simulink model "chip_route_iso_mdl"  (R2025b)
settings: Solver=VariableStepAuto  StartTime=0.0  StopTime=10.0  RelTol=1e-3
libraries: fl_lib x62, nesl_utility x1
settings Model: Creator=97638  LastModifiedBy=97638

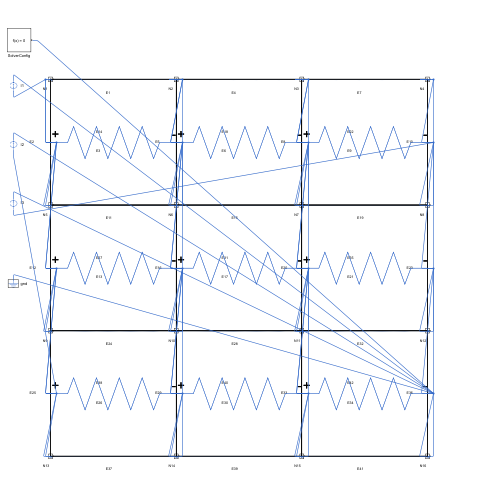
[thumbnail: Simulink's stored preview of the top-level diagram]
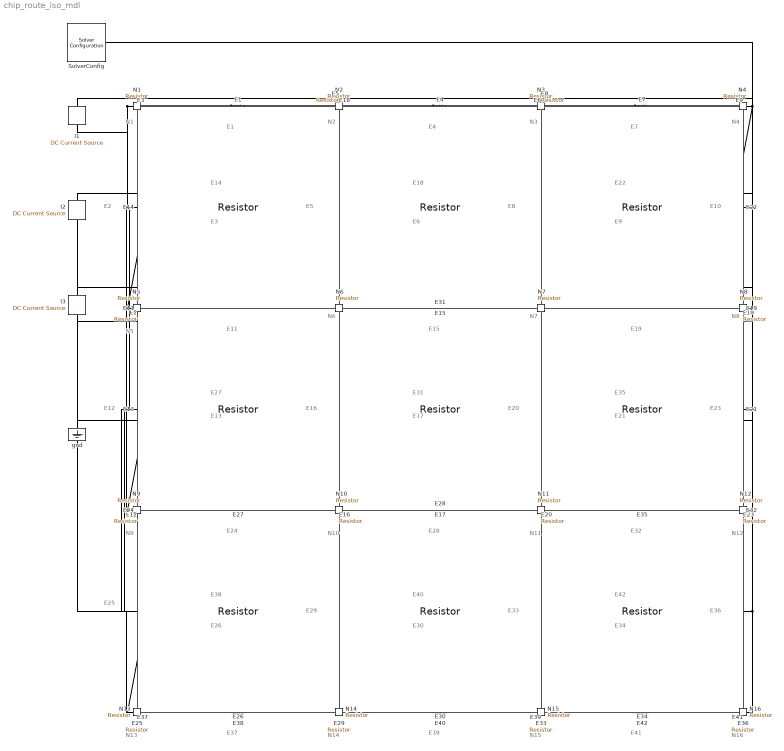
== system chip_route_iso_mdl ==
  note: N1
  note: N2
  note: N3
  note: N4
  note: N5
  note: N6
  note: N7
  note: N8
  note: N9
  note: N10
  note: N11
  note: N12
  note: N13
  note: N14
  note: N15
  note: N16
  note: E1
  note: E2
  note: E3
  note: E4
  note: E5
  note: E6
  note: E7
  note: E8
  note: E9
  note: E10
  note: E11
  note: E12
  note: E13
  note: E14
  note: E15
  note: E16
  note: E17
  note: E18
  note: E19
  note: E20
  note: E21
  note: E22
  note: E23
  note: E24
  note: E25
  note: E26
  note: E27
  note: E28
  note: E29
  note: E30
  note: E31
  note: E32
  note: E33
  note: E34
  note: E35
  note: E36
  note: E37
  note: E38
  note: E39
  note: E40
  note: E41
  note: E42
  E{1..2,4..5,7..8,10..12,15..16,19..20,23..25,28..29,32..33,36..37,39,41} (24 alike) : fl_lib/Electrical/Electrical Elements/Resistor  R=1.000000 Ohm  i_specify=off  i_priority=None  i=0 A  i_nominal_specify=off  i_nominal_value=1  i_nominal_unit=A  v_specify=off  v_priority=None  v=0 V  v_nominal_specify=off  v_nominal_value=1  v_nominal_unit=V  mask(Resistor){}
      E1 mask Display:
      | line([0.0000,0.2500],[0.5000,0.5000]);
      | line([0.2500,0.3125,0.3750,0.4375,0.5000,0.5625,0.6250,0.6875,0.7500],[0.5000,0.4000,0.6000,0.4000,0.6000,0.4000,0.6000,0.4000,0.5000]);
      | line([0.7500,1.0000],[0.5000,0.5000]);
      E10 mask Display:
      | line([0.5000,0.5000],[0.0000,0.2500]);
      | line([0.5000,0.6000,0.4000,0.6000,0.4000,0.6000,0.4000,0.6000,0.5000],[0.2500,0.3125,0.3750,0.4375,0.5000,0.5625,0.6250,0.6875,0.7500]);
      | line([0.5000,0.5000],[0.7500,1.0000]);
      E11 mask Display:
      | line([0.0000,0.2500],[0.5000,0.5000]);
      | line([0.2500,0.3125,0.3750,0.4375,0.5000,0.5625,0.6250,0.6875,0.7500],[0.5000,0.4000,0.6000,0.4000,0.6000,0.4000,0.6000,0.4000,0.5000]);
      | line([0.7500,1.0000],[0.5000,0.5000]);
      E12 mask Display:
      | line([0.5000,0.5000],[0.0000,0.2500]);
      | line([0.5000,0.6000,0.4000,0.6000,0.4000,0.6000,0.4000,0.6000,0.5000],[0.2500,0.3125,0.3750,0.4375,0.5000,0.5625,0.6250,0.6875,0.7500]);
      | line([0.5000,0.5000],[0.7500,1.0000]);
      E15 mask Display:
      | line([0.0000,0.2500],[0.5000,0.5000]);
      | line([0.2500,0.3125,0.3750,0.4375,0.5000,0.5625,0.6250,0.6875,0.7500],[0.5000,0.4000,0.6000,0.4000,0.6000,0.4000,0.6000,0.4000,0.5000]);
      | line([0.7500,1.0000],[0.5000,0.5000]);
      E16 mask Display:
      | line([0.5000,0.5000],[0.0000,0.2500]);
      | line([0.5000,0.6000,0.4000,0.6000,0.4000,0.6000,0.4000,0.6000,0.5000],[0.2500,0.3125,0.3750,0.4375,0.5000,0.5625,0.6250,0.6875,0.7500]);
      | line([0.5000,0.5000],[0.7500,1.0000]);
      E19 mask Display:
      | line([0.0000,0.2500],[0.5000,0.5000]);
      | line([0.2500,0.3125,0.3750,0.4375,0.5000,0.5625,0.6250,0.6875,0.7500],[0.5000,0.4000,0.6000,0.4000,0.6000,0.4000,0.6000,0.4000,0.5000]);
      | line([0.7500,1.0000],[0.5000,0.5000]);
      E2 mask Display:
      | line([0.5000,0.5000],[0.0000,0.2500]);
      | line([0.5000,0.6000,0.4000,0.6000,0.4000,0.6000,0.4000,0.6000,0.5000],[0.2500,0.3125,0.3750,0.4375,0.5000,0.5625,0.6250,0.6875,0.7500]);
      | line([0.5000,0.5000],[0.7500,1.0000]);
      E20 mask Display:
      | line([0.5000,0.5000],[0.0000,0.2500]);
      | line([0.5000,0.6000,0.4000,0.6000,0.4000,0.6000,0.4000,0.6000,0.5000],[0.2500,0.3125,0.3750,0.4375,0.5000,0.5625,0.6250,0.6875,0.7500]);
      | line([0.5000,0.5000],[0.7500,1.0000]);
      E23 mask Display:
      | line([0.5000,0.5000],[0.0000,0.2500]);
      | line([0.5000,0.6000,0.4000,0.6000,0.4000,0.6000,0.4000,0.6000,0.5000],[0.2500,0.3125,0.3750,0.4375,0.5000,0.5625,0.6250,0.6875,0.7500]);
      | line([0.5000,0.5000],[0.7500,1.0000]);
      E24 mask Display:
      | line([0.0000,0.2500],[0.5000,0.5000]);
      | line([0.2500,0.3125,0.3750,0.4375,0.5000,0.5625,0.6250,0.6875,0.7500],[0.5000,0.4000,0.6000,0.4000,0.6000,0.4000,0.6000,0.4000,0.5000]);
      | line([0.7500,1.0000],[0.5000,0.5000]);
      E25 mask Display:
      | line([0.5000,0.5000],[0.0000,0.2500]);
      | line([0.5000,0.6000,0.4000,0.6000,0.4000,0.6000,0.4000,0.6000,0.5000],[0.2500,0.3125,0.3750,0.4375,0.5000,0.5625,0.6250,0.6875,0.7500]);
      | line([0.5000,0.5000],[0.7500,1.0000]);
      E28 mask Display:
      | line([0.0000,0.2500],[0.5000,0.5000]);
      | line([0.2500,0.3125,0.3750,0.4375,0.5000,0.5625,0.6250,0.6875,0.7500],[0.5000,0.4000,0.6000,0.4000,0.6000,0.4000,0.6000,0.4000,0.5000]);
      | line([0.7500,1.0000],[0.5000,0.5000]);
      E29 mask Display:
      | line([0.5000,0.5000],[0.0000,0.2500]);
      | line([0.5000,0.6000,0.4000,0.6000,0.4000,0.6000,0.4000,0.6000,0.5000],[0.2500,0.3125,0.3750,0.4375,0.5000,0.5625,0.6250,0.6875,0.7500]);
      | line([0.5000,0.5000],[0.7500,1.0000]);
      E32 mask Display:
      | line([0.0000,0.2500],[0.5000,0.5000]);
      | line([0.2500,0.3125,0.3750,0.4375,0.5000,0.5625,0.6250,0.6875,0.7500],[0.5000,0.4000,0.6000,0.4000,0.6000,0.4000,0.6000,0.4000,0.5000]);
      | line([0.7500,1.0000],[0.5000,0.5000]);
      E33 mask Display:
      | line([0.5000,0.5000],[0.0000,0.2500]);
      | line([0.5000,0.6000,0.4000,0.6000,0.4000,0.6000,0.4000,0.6000,0.5000],[0.2500,0.3125,0.3750,0.4375,0.5000,0.5625,0.6250,0.6875,0.7500]);
      | line([0.5000,0.5000],[0.7500,1.0000]);
      E36 mask Display:
      | line([0.5000,0.5000],[0.0000,0.2500]);
      | line([0.5000,0.6000,0.4000,0.6000,0.4000,0.6000,0.4000,0.6000,0.5000],[0.2500,0.3125,0.3750,0.4375,0.5000,0.5625,0.6250,0.6875,0.7500]);
      | line([0.5000,0.5000],[0.7500,1.0000]);
      E37 mask Display:
      | line([0.0000,0.2500],[0.5000,0.5000]);
      | line([0.2500,0.3125,0.3750,0.4375,0.5000,0.5625,0.6250,0.6875,0.7500],[0.5000,0.4000,0.6000,0.4000,0.6000,0.4000,0.6000,0.4000,0.5000]);
      | line([0.7500,1.0000],[0.5000,0.5000]);
      E39 mask Display:
      | line([0.0000,0.2500],[0.5000,0.5000]);
      | line([0.2500,0.3125,0.3750,0.4375,0.5000,0.5625,0.6250,0.6875,0.7500],[0.5000,0.4000,0.6000,0.4000,0.6000,0.4000,0.6000,0.4000,0.5000]);
      | line([0.7500,1.0000],[0.5000,0.5000]);
      E4 mask Display:
      | line([0.0000,0.2500],[0.5000,0.5000]);
      | line([0.2500,0.3125,0.3750,0.4375,0.5000,0.5625,0.6250,0.6875,0.7500],[0.5000,0.4000,0.6000,0.4000,0.6000,0.4000,0.6000,0.4000,0.5000]);
      | line([0.7500,1.0000],[0.5000,0.5000]);
      E41 mask Display:
      | line([0.0000,0.2500],[0.5000,0.5000]);
      | line([0.2500,0.3125,0.3750,0.4375,0.5000,0.5625,0.6250,0.6875,0.7500],[0.5000,0.4000,0.6000,0.4000,0.6000,0.4000,0.6000,0.4000,0.5000]);
      | line([0.7500,1.0000],[0.5000,0.5000]);
      E5 mask Display:
      | line([0.5000,0.5000],[0.0000,0.2500]);
      | line([0.5000,0.6000,0.4000,0.6000,0.4000,0.6000,0.4000,0.6000,0.5000],[0.2500,0.3125,0.3750,0.4375,0.5000,0.5625,0.6250,0.6875,0.7500]);
      | line([0.5000,0.5000],[0.7500,1.0000]);
      E7 mask Display:
      | line([0.0000,0.2500],[0.5000,0.5000]);
      | line([0.2500,0.3125,0.3750,0.4375,0.5000,0.5625,0.6250,0.6875,0.7500],[0.5000,0.4000,0.6000,0.4000,0.6000,0.4000,0.6000,0.4000,0.5000]);
      | line([0.7500,1.0000],[0.5000,0.5000]);
      E8 mask Display:
      | line([0.5000,0.5000],[0.0000,0.2500]);
      | line([0.5000,0.6000,0.4000,0.6000,0.4000,0.6000,0.4000,0.6000,0.5000],[0.2500,0.3125,0.3750,0.4375,0.5000,0.5625,0.6250,0.6875,0.7500]);
      | line([0.5000,0.5000],[0.7500,1.0000]);
  E{3,6,9,13..14,17..18,21..22,26..27,30..31,34..35,38,40,42} (18 alike) : fl_lib/Electrical/Electrical Elements/Resistor  R=1.414214 Ohm  i_specify=off  i_priority=None  i=0 A  i_nominal_specify=off  i_nominal_value=1  i_nominal_unit=A  v_specify=off  v_priority=None  v=0 V  v_nominal_specify=off  v_nominal_value=1  v_nominal_unit=V  mask(Resistor){}
      E13 mask Display:
      | line([0.0000,0.2500],[0.0000,0.2500]);
      | line([0.2500,0.3832,0.3043,0.5082,0.4293,0.6332,0.5543,0.7582,0.7500],[0.2500,0.2418,0.4457,0.3668,0.5707,0.4918,0.6957,0.6168,0.7500]);
      | line([0.7500,1.0000],[0.7500,1.0000]);
      E14 mask Display:
      | line([0.0000,0.2500],[1.0000,0.7500]);
      | line([0.2500,0.2418,0.4457,0.3668,0.5707,0.4918,0.6957,0.6168,0.7500],[0.7500,0.6168,0.6957,0.4918,0.5707,0.3668,0.4457,0.2418,0.2500]);
      | line([0.7500,1.0000],[0.2500,0.0000]);
      E17 mask Display:
      | line([0.0000,0.2500],[0.0000,0.2500]);
      | line([0.2500,0.3832,0.3043,0.5082,0.4293,0.6332,0.5543,0.7582,0.7500],[0.2500,0.2418,0.4457,0.3668,0.5707,0.4918,0.6957,0.6168,0.7500]);
      | line([0.7500,1.0000],[0.7500,1.0000]);
      E18 mask Display:
      | line([0.0000,0.2500],[1.0000,0.7500]);
      | line([0.2500,0.2418,0.4457,0.3668,0.5707,0.4918,0.6957,0.6168,0.7500],[0.7500,0.6168,0.6957,0.4918,0.5707,0.3668,0.4457,0.2418,0.2500]);
      | line([0.7500,1.0000],[0.2500,0.0000]);
      E21 mask Display:
      | line([0.0000,0.2500],[0.0000,0.2500]);
      | line([0.2500,0.3832,0.3043,0.5082,0.4293,0.6332,0.5543,0.7582,0.7500],[0.2500,0.2418,0.4457,0.3668,0.5707,0.4918,0.6957,0.6168,0.7500]);
      | line([0.7500,1.0000],[0.7500,1.0000]);
      E22 mask Display:
      | line([0.0000,0.2500],[1.0000,0.7500]);
      | line([0.2500,0.2418,0.4457,0.3668,0.5707,0.4918,0.6957,0.6168,0.7500],[0.7500,0.6168,0.6957,0.4918,0.5707,0.3668,0.4457,0.2418,0.2500]);
      | line([0.7500,1.0000],[0.2500,0.0000]);
      E26 mask Display:
      | line([0.0000,0.2500],[0.0000,0.2500]);
      | line([0.2500,0.3832,0.3043,0.5082,0.4293,0.6332,0.5543,0.7582,0.7500],[0.2500,0.2418,0.4457,0.3668,0.5707,0.4918,0.6957,0.6168,0.7500]);
      | line([0.7500,1.0000],[0.7500,1.0000]);
      E27 mask Display:
      | line([0.0000,0.2500],[1.0000,0.7500]);
      | line([0.2500,0.2418,0.4457,0.3668,0.5707,0.4918,0.6957,0.6168,0.7500],[0.7500,0.6168,0.6957,0.4918,0.5707,0.3668,0.4457,0.2418,0.2500]);
      | line([0.7500,1.0000],[0.2500,0.0000]);
      E3 mask Display:
      | line([0.0000,0.2500],[0.0000,0.2500]);
      | line([0.2500,0.3832,0.3043,0.5082,0.4293,0.6332,0.5543,0.7582,0.7500],[0.2500,0.2418,0.4457,0.3668,0.5707,0.4918,0.6957,0.6168,0.7500]);
      | line([0.7500,1.0000],[0.7500,1.0000]);
      E30 mask Display:
      | line([0.0000,0.2500],[0.0000,0.2500]);
      | line([0.2500,0.3832,0.3043,0.5082,0.4293,0.6332,0.5543,0.7582,0.7500],[0.2500,0.2418,0.4457,0.3668,0.5707,0.4918,0.6957,0.6168,0.7500]);
      | line([0.7500,1.0000],[0.7500,1.0000]);
      E31 mask Display:
      | line([0.0000,0.2500],[1.0000,0.7500]);
      | line([0.2500,0.2418,0.4457,0.3668,0.5707,0.4918,0.6957,0.6168,0.7500],[0.7500,0.6168,0.6957,0.4918,0.5707,0.3668,0.4457,0.2418,0.2500]);
      | line([0.7500,1.0000],[0.2500,0.0000]);
      E34 mask Display:
      | line([0.0000,0.2500],[0.0000,0.2500]);
      | line([0.2500,0.3832,0.3043,0.5082,0.4293,0.6332,0.5543,0.7582,0.7500],[0.2500,0.2418,0.4457,0.3668,0.5707,0.4918,0.6957,0.6168,0.7500]);
      | line([0.7500,1.0000],[0.7500,1.0000]);
      E35 mask Display:
      | line([0.0000,0.2500],[1.0000,0.7500]);
      | line([0.2500,0.2418,0.4457,0.3668,0.5707,0.4918,0.6957,0.6168,0.7500],[0.7500,0.6168,0.6957,0.4918,0.5707,0.3668,0.4457,0.2418,0.2500]);
      | line([0.7500,1.0000],[0.2500,0.0000]);
      E38 mask Display:
      | line([0.0000,0.2500],[1.0000,0.7500]);
      | line([0.2500,0.2418,0.4457,0.3668,0.5707,0.4918,0.6957,0.6168,0.7500],[0.7500,0.6168,0.6957,0.4918,0.5707,0.3668,0.4457,0.2418,0.2500]);
      | line([0.7500,1.0000],[0.2500,0.0000]);
      E40 mask Display:
      | line([0.0000,0.2500],[1.0000,0.7500]);
      | line([0.2500,0.2418,0.4457,0.3668,0.5707,0.4918,0.6957,0.6168,0.7500],[0.7500,0.6168,0.6957,0.4918,0.5707,0.3668,0.4457,0.2418,0.2500]);
      | line([0.7500,1.0000],[0.2500,0.0000]);
      E42 mask Display:
      | line([0.0000,0.2500],[1.0000,0.7500]);
      | line([0.2500,0.2418,0.4457,0.3668,0.5707,0.4918,0.6957,0.6168,0.7500],[0.7500,0.6168,0.6957,0.4918,0.5707,0.3668,0.4457,0.2418,0.2500]);
      | line([0.7500,1.0000],[0.2500,0.0000]);
      E6 mask Display:
      | line([0.0000,0.2500],[0.0000,0.2500]);
      | line([0.2500,0.3832,0.3043,0.5082,0.4293,0.6332,0.5543,0.7582,0.7500],[0.2500,0.2418,0.4457,0.3668,0.5707,0.4918,0.6957,0.6168,0.7500]);
      | line([0.7500,1.0000],[0.7500,1.0000]);
      E9 mask Display:
      | line([0.0000,0.2500],[0.0000,0.2500]);
      | line([0.2500,0.3832,0.3043,0.5082,0.4293,0.6332,0.5543,0.7582,0.7500],[0.2500,0.2418,0.4457,0.3668,0.5707,0.4918,0.6957,0.6168,0.7500]);
      | line([0.7500,1.0000],[0.7500,1.0000]);
  I1 : fl_lib/Electrical/Electrical Sources/DC Current Source  i0=1.0000 A
      settings: InternalSimscapePortConfiguration="{\"Bottom\":[],\"Left\":[{\"id\":\"p\",\"label\":\"\",\"type\":\"foundation.electrical.electrical\"}],\"Right\":[{\"id\":\"n\",\"label\":\"\",\"type\":\"foundation.electrical.electrical\"}],\"Top\":[]}"
  I2 : fl_lib/Electrical/Electrical Sources/DC Current Source  i0=1.0000 A
      settings: InternalSimscapePortConfiguration="{\"Bottom\":[],\"Left\":[{\"id\":\"p\",\"label\":\"\",\"type\":\"foundation.electrical.electrical\"}],\"Right\":[{\"id\":\"n\",\"label\":\"\",\"type\":\"foundation.electrical.electrical\"}],\"Top\":[]}"
  I3 : fl_lib/Electrical/Electrical Sources/DC Current Source  i0=-2.0000 A
      settings: InternalSimscapePortConfiguration="{\"Bottom\":[],\"Left\":[{\"id\":\"p\",\"label\":\"\",\"type\":\"foundation.electrical.electrical\"}],\"Right\":[{\"id\":\"n\",\"label\":\"\",\"type\":\"foundation.electrical.electrical\"}],\"Top\":[]}"
  N{1..16} (16 alike) : fl_lib/Electrical/Electrical Elements/Resistor  R=1e-6 Ohm  i_specify=off  i_priority=None  i=0 A  i_nominal_specify=off  i_nominal_value=1  i_nominal_unit=A  v_specify=off  v_priority=None  v=0 V  v_nominal_specify=off  v_nominal_value=1  v_nominal_unit=V  mask(Resistor){}
      mask Display: line([0.42,0.58],[0.5,0.5]);line([0.5,0.5],[0.42,0.58]);
  SolverConfig : nesl_utility/Solver Configuration  PhysicalDomain=network_engine_domain  SubClassName=solver  LeftPortType=input  RightPortType=generic  Tones=[]  Harmonics=[]  SimulateNoise=off  Profile=off  UseLocalSampling=off  EnableSwitchedLinearOptims=on  FrequencyDomain=off  UseCCode=off  RelTol=0.001  AbsTol=0.001  MinStep=1e-09  ToWorkspace=off  RevertToSquareIcSolve=off  NumHomotopyIterations=100  PhasorMode=off  PhasorModeNumHarmonics=1  ConsistencySolver=NEWTON_XTOL_AFTER_FTOL  IndexReductionMethod=DerivativeReplacement  DoDC=off  ResidualTolerance=1e-09  ConsistencyTolSource=GLOBAL  ConsistencyAbsTol=0.001  ConsistencyRelTol=0.001  ConsistencyTolFactor=0.001  UseLocalSolver=off  LocalSolverChoice=NE_BACKWARD_EULER_ADVANCER  ResolveIndetEquations=on  FunctionEvalNumThread=1  LocalSolverSampleTime=0.001  DoFixedCost=off  MaxNonlinIter=3  MaxModeIter=2  ComputeImpulses=off  ImpulseIterations=2  LinearAlgebra=auto  LinearAlgebraNumThread=0  EquationFormulation=NE_TIME_EF  DelaysMemoryBudget=1024  AutomaticFiltering=on  FilteringTimeConstant=0.001  PartitionStorageMethod=AS_NEEDED  PartitionMemoryBudget=1024  PartitionMethod=ROBUST  MultibodyUseLocalSolver=off  MultibodyLocalSolverChoice=ODE1  MultibodyLocalSolverSampleTime=0.001
  gnd : fl_lib/Electrical/Electrical Elements/Electrical Reference
  connections:
  E2/LConn1 -- E1/LConn1 -- E3/LConn1 -- N1/LConn1 -- I1/RConn1
  E4/LConn1 -- E1/RConn1 -- E5/LConn1 -- E6/LConn1 -- E14/RConn1 -- N2/LConn1
  E7/LConn1 -- E4/RConn1 -- E8/LConn1 -- E9/LConn1 -- E18/RConn1 -- N3/LConn1
  E10/LConn1 -- E7/RConn1 -- E22/RConn1 -- N4/LConn1
  E11/LConn1 -- E2/RConn1 -- E12/LConn1 -- E13/LConn1 -- E14/LConn1 -- N5/LConn1
  E5/RConn1 -- E3/RConn1 -- E11/RConn1 -- E15/LConn1 -- E16/LConn1 -- E17/LConn1 -- E18/LConn1 -- E27/RConn1 -- N6/LConn1
  E8/RConn1 -- E6/RConn1 -- E15/RConn1 -- E19/LConn1 -- E20/LConn1 -- E21/LConn1 -- E22/LConn1 -- E31/RConn1 -- N7/LConn1
  E10/RConn1 -- E9/RConn1 -- E19/RConn1 -- E23/LConn1 -- E35/RConn1 -- N8/LConn1 -- I3/RConn1
  E24/LConn1 -- E12/RConn1 -- E25/LConn1 -- E26/LConn1 -- E27/LConn1 -- N9/LConn1
  E16/RConn1 -- E13/RConn1 -- E24/RConn1 -- E28/LConn1 -- E29/LConn1 -- E30/LConn1 -- E31/LConn1 -- E38/RConn1 -- N10/LConn1
  E20/RConn1 -- E17/RConn1 -- E28/RConn1 -- E32/LConn1 -- E33/LConn1 -- E34/LConn1 -- E35/LConn1 -- E40/RConn1 -- N11/LConn1
  E23/RConn1 -- E21/RConn1 -- E32/RConn1 -- E36/LConn1 -- E42/RConn1 -- N12/LConn1
  E37/LConn1 -- E25/RConn1 -- E38/LConn1 -- N13/LConn1 -- I2/RConn1
  E29/RConn1 -- E26/RConn1 -- E37/RConn1 -- E39/LConn1 -- E40/LConn1 -- N14/LConn1
  E33/RConn1 -- E30/RConn1 -- E39/RConn1 -- E41/LConn1 -- E42/LConn1 -- N15/LConn1
  E36/RConn1 -- E34/RConn1 -- E41/RConn1 -- N16/LConn1 -- gnd/LConn1 -- I1/LConn1 -- I2/LConn1 -- I3/LConn1 -- SolverConfig/RConn1
